simulink model "can2_comp_cmd_pack"  (R2026b)
settings: Solver=VariableStepAuto
undefined symbols (not defined in the file or in its folder): P
libraries: simulink x1, svdutilitieslib x1
settings Model: Creator=aomar  LastModifiedBy=aomar

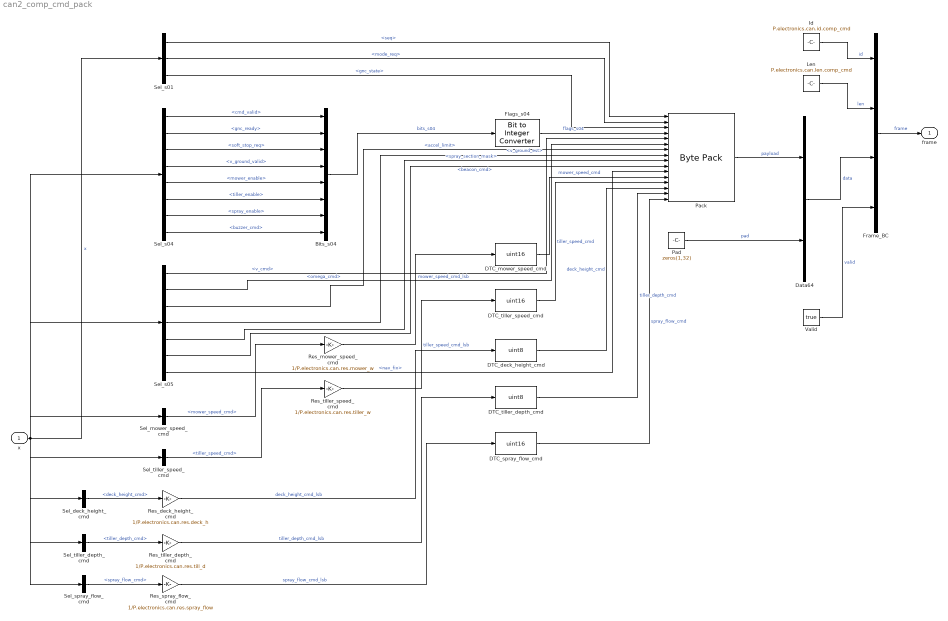
== system can2_comp_cmd_pack ==
  x : Inport  OutDataTypeStr=Bus: Bus_GncCmd
  Bits_s04 : Concatenate  NumInputs=8
  DTC_deck_height_cmd : DataTypeConversion  OutDataTypeStr=uint8  RndMeth=Round
  DTC_mower_speed_cmd : DataTypeConversion  OutDataTypeStr=uint16  RndMeth=Round
  DTC_spray_flow_cmd : DataTypeConversion  OutDataTypeStr=uint16  RndMeth=Round
  DTC_tiller_depth_cmd : DataTypeConversion  OutDataTypeStr=uint8  RndMeth=Round
  DTC_tiller_speed_cmd : DataTypeConversion  OutDataTypeStr=uint16  RndMeth=Round
  Data64 : Concatenate
  Flags_s04 : simulink/Logic and Bit Operations/Bit to Integer Converter  nbits=8  bitOrder=LSB first  signedOutputValues=Unsigned  outDtype=uint8  outDtypeSigned=Inherit via internal rule
      settings: LibrarySourceBlock=|
      | commutil2/Bit to Integer
      | Converter
  Frame_BC : BusCreator  Inputs=4  OutDataTypeStr=Bus: Bus_CanFrame64  NonVirtualBus=on
      settings: InheritFromInputs=off
  Id : Constant  Value=P.electronics.can.id.comp_cmd  OutDataTypeStr=uint32  SampleTime=-1
  Len : Constant  Value=P.electronics.can.len.comp_cmd  OutDataTypeStr=uint8  SampleTime=-1
  Pack : svdutilitieslib/Byte Pack  maskPackedDataType=uint8  datatypes={'uint8','uint8','uint8','uint8','single','single','single','single','uint16','uint8','uint8','uint16','uint16','uint8','uint8','uint16'}  byteAlign=1  blockPlatform=arduinoert
      settings: LibrarySourceBlock=mcblib/Signal Management/Byte Pack
  Pad : Constant  Value=zeros(1,32)  OutDataTypeStr=uint8  SampleTime=-1
  Res_deck_height_cmd : Gain  Gain=1/P.electronics.can.res.deck_h
  Res_mower_speed_cmd : Gain  Gain=1/P.electronics.can.res.mower_w
  Res_spray_flow_cmd : Gain  Gain=1/P.electronics.can.res.spray_flow
  Res_tiller_depth_cmd : Gain  Gain=1/P.electronics.can.res.till_d
  Res_tiller_speed_cmd : Gain  Gain=1/P.electronics.can.res.tiller_w
  Sel_deck_height_cmd : BusSelector  OutputSignals=deck_height_cmd
  Sel_mower_speed_cmd : BusSelector  OutputSignals=mower_speed_cmd
  Sel_s01 : BusSelector  OutputSignals=seq,mode_req,gnc_state
  Sel_s04 : BusSelector  OutputSignals=cmd_valid,gnc_ready,soft_stop_req,v_ground_valid,mower_enable,tiller_enable,spray_enable,buzzer_cmd
  Sel_s05 : BusSelector  OutputSignals=v_cmd,omega_cmd,accel_limit,v_ground_est,spray_section_mask,beacon_cmd,nav_fix
  Sel_spray_flow_cmd : BusSelector  OutputSignals=spray_flow_cmd
  Sel_tiller_depth_cmd : BusSelector  OutputSignals=tiller_depth_cmd
  Sel_tiller_speed_cmd : BusSelector  OutputSignals=tiller_speed_cmd
  Valid : Constant  Value=true  OutDataTypeStr=boolean  SampleTime=-1
  frame : Outport  OutDataTypeStr=Bus: Bus_CanFrame64
  wires:
  x/1 -> Sel_s01/1, Sel_s04/1, Sel_spray_flow_cmd/1, Sel_s05/1, Sel_tiller_depth_cmd/1, Sel_deck_height_cmd/1, Sel_mower_speed_cmd/1, Sel_tiller_speed_cmd/1  "x"
  Sel_deck_height_cmd/1 -> Res_deck_height_cmd/1  "<deck_height_cmd>"
  Sel_tiller_depth_cmd/1 -> Res_tiller_depth_cmd/1  "<tiller_depth_cmd>"
  Sel_spray_flow_cmd/1 -> Res_spray_flow_cmd/1  "<spray_flow_cmd>"
  Sel_s01/1 -> Pack/1  "<seq>"
  Sel_s01/2 -> Pack/2  "<mode_req>"
  Sel_s01/3 -> Pack/3  "<gnc_state>"
  Sel_s04/1 -> Bits_s04/1  "<cmd_valid>"
  Sel_s04/2 -> Bits_s04/2  "<gnc_ready>"
  Sel_s04/3 -> Bits_s04/3  "<soft_stop_req>"
  Sel_s04/4 -> Bits_s04/4  "<v_ground_valid>"
  Sel_s04/5 -> Bits_s04/5  "<mower_enable>"
  Sel_s04/6 -> Bits_s04/6  "<tiller_enable>"
  Sel_s04/7 -> Bits_s04/7  "<spray_enable>"
  Sel_s04/8 -> Bits_s04/8  "<buzzer_cmd>"
  Sel_s05/1 -> Pack/5  "<v_cmd>"
  Sel_s05/2 -> Pack/6  "<omega_cmd>"
  Sel_s05/3 -> Pack/7  "<accel_limit>"
  Sel_s05/4 -> Pack/8  "<v_ground_est>"
  Sel_s05/5 -> Pack/9  "<spray_section_mask>"
  Sel_s05/6 -> Pack/10  "<beacon_cmd>"
  Sel_s05/7 -> Pack/11  "<nav_fix>"
  Sel_mower_speed_cmd/1 -> Res_mower_speed_cmd/1  "<mower_speed_cmd>"
  Sel_tiller_speed_cmd/1 -> Res_tiller_speed_cmd/1  "<tiller_speed_cmd>"
  Res_deck_height_cmd/1 -> DTC_deck_height_cmd/1  "deck_height_cmd_lsb"
  Res_tiller_depth_cmd/1 -> DTC_tiller_depth_cmd/1  "tiller_depth_cmd_lsb"
  Res_spray_flow_cmd/1 -> DTC_spray_flow_cmd/1  "spray_flow_cmd_lsb"
  Bits_s04/1 -> Flags_s04/1  "bits_s04"
  Res_mower_speed_cmd/1 -> DTC_mower_speed_cmd/1  "mower_speed_cmd_lsb"
  Res_tiller_speed_cmd/1 -> DTC_tiller_speed_cmd/1  "tiller_speed_cmd_lsb"
  DTC_mower_speed_cmd/1 -> Pack/12  "mower_speed_cmd"
  DTC_tiller_speed_cmd/1 -> Pack/13  "tiller_speed_cmd"
  DTC_deck_height_cmd/1 -> Pack/14  "deck_height_cmd"
  DTC_tiller_depth_cmd/1 -> Pack/15  "tiller_depth_cmd"
  DTC_spray_flow_cmd/1 -> Pack/16  "spray_flow_cmd"
  Flags_s04/1 -> Pack/4  "flags_s04"
  Pad/1 -> Data64/2  "pad"
  Pack/1 -> Data64/1  "payload"
  Data64/1 -> Frame_BC/3  "data"
  Id/1 -> Frame_BC/1  "id"
  Len/1 -> Frame_BC/2  "len"
  Valid/1 -> Frame_BC/4  "valid"
  Frame_BC/1 -> frame/1  "frame"
